simulink model ""  (R2026a)
settings: Solver=FixedStepDiscrete  StopTime=Inf  FixedStep=0.01
PreLoadFcn:
  | rbt = exampleHelperSetUpCobot();
  | 
  | %maxNumOfBoxes = 30;
  | %boxDim = 0.2;
  | %boxPosition = [-0.65 0.45 0.6];
  | 
  | % initSim.m
  | data = readmatrix('boxes.xlsx');  % Now it's a double matrix
  | boxDim = data(1, 2:4);
  | boxPosition = data(1, 6:8);
  | maxNumOfBoxes = length(data(:,1));
  | boxWeight = data(1,5);
  | assignin('base', 'data', data);
  | assignin('base', 'boxDim', boxDim);
  | assignin('base', 'boxPosition', boxPosition);
InitFcn:
  | data = readmatrix('boxes.xlsx');  % Now it's a double matrix
  | boxDim = data(1, 2:4);
  | boxPosition = data(1, 6:8);
  | maxNumOfBoxes = length(data(:,1));
  | boxWeight = data(1,5);
StartFcn:
  | coder.extrinsic("spawnBox")
  | 
  | % Spawn the first box on the bench
  | K = [0.2, 0.2, 0.2];
  | Wt = 0.2;
  | spawnBox(0, boxPosition, boxDim, boxWeight)
libraries: sim3dlib x2, robotcorelib x2, robotmaniplib x2, robotsim3dlib x1
settings Model: PauseTimes=1  Creator=araman  LastModifiedBy=fofr6825
settings DebuggingCC: ReadBeforeWriteMsg=DisableAll  WriteAfterWriteMsg=DisableAll  WriteAfterReadMsg=DisableAll  MultiTaskDSMMsg=none
settings SFSimCC: SFSimEcho=off
settings SimscapeCC: SimscapeNominalValues="[{\"value\":\"1\",\"unit\":\"A\"},{\"value\":\"1\",\"unit\":\"bar\"},{\"value\":\"1\",\"unit\":\"cm^2\"},{\"value\":\"1\",\"unit\":\"cm^3/s\"},{\"value\":\"1\",\"unit\":\"kJ/kg\"},{\"value\":\"1\",\"unit\":\"kW\"},{\"value\":\"1\",\"unit\":\"l\"},{\"value\":\"1\",\"unit\":\"N\"},{\"value\":\"1\",\"unit\":\"N*m\"},{\"value\":\"1\",\"unit\":\"V\"}]"  SimscapeLogType=none  SimscapeLogDataHistory=5000.0

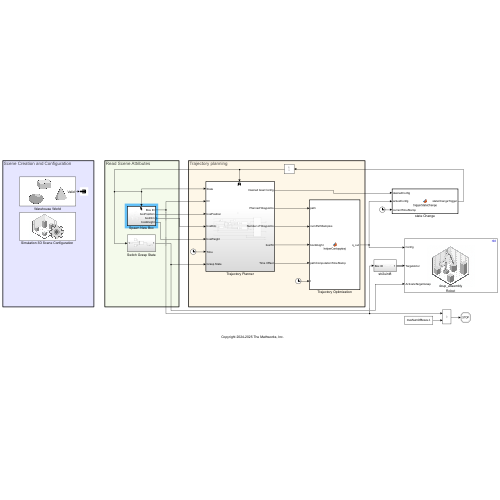
[thumbnail: Simulink's stored preview of the top-level diagram]
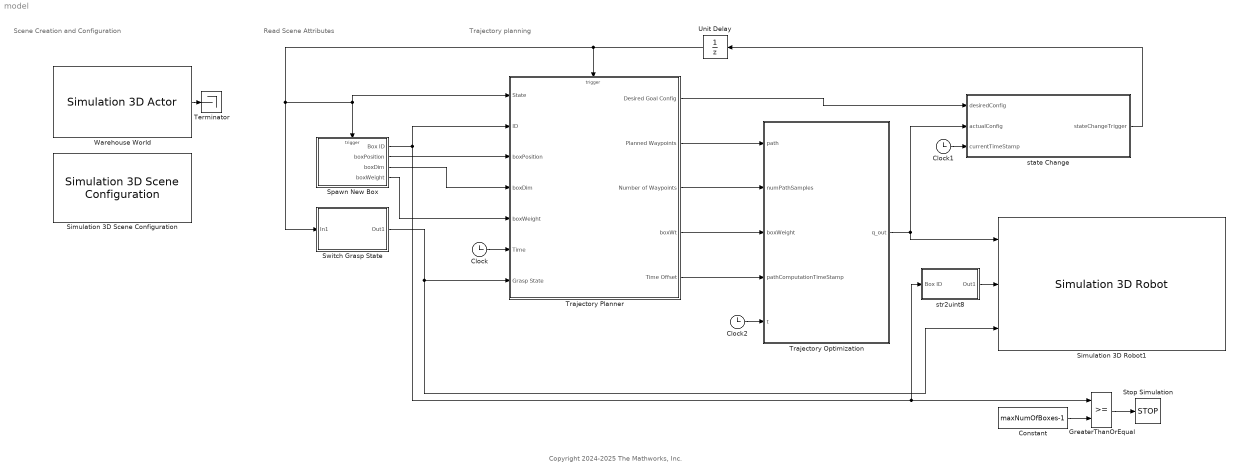
== system model ==
  note: Copyright 2024-2025 The Mathworks, Inc.
  note: Trajectory planning
  note: Scene Creation and Configuration
  note: Read Scene Attributes
  Clock : Clock
  Clock1 : Clock
  Clock2 : Clock
  Constant : Constant  Value=maxNumOfBoxes-1
  GreaterThanOrEqual : RelationalOperator  OutDataTypeStr=boolean  RndMeth=Simplest  InputSameDT=off
  Simulation 3D Robot1 : robotsim3dlib/Simulation 3D Robot  actorInputType=RigidBodyTree Object  RigidBodyTree=rbt  ActorName=Robot  existActorChekBox=off  initialTrans=[0 0 0]  initialRot=[0 0 0]  initialConfig="[2.8471   -1.6598    2.1329    4.2393   -1.5708    4.4179]"  EndEffector=4cup_assembly  eeOffsetInpChekBox=off  eeTargetTrans=[0 -0.2 0]  eeTargetRot=[0 0 0]  enableRegionGraspChekBox=off  regionGraspInpChekBox=off  eeTargTransDiff=[0.2 0.2 0.2]  eeTargRotDiff=[0 0 0]  enableVisualVisualization=on  enableCollisionVisualization=off  collisionGeomColor=[0 1 0]  collisionGeomTransp=0.1  inpConfEnbVal=on  inpGraspEnbVal=on  inpTransEnbVal=off  outConfEnbVal=off  outGraspEnbVal=off  outTransEnbVal=off  SampleTime=-1  ActorType=SimulinkVehicle  ID=C  aMode=6  ActorTag=Robot  Mesh=RigidBodyTree
  "Simulation 3D Scene Configuration " : sim3dlib/Simulation 3D Scene Configuration  Priority=0  ProjectFormat=Default Scenes  SceneDesc=Empty scene  ProjectName=C:\Program Files\MATLAB\R2026a\toolbox\shared\sim3d_projects\automotive_project_windows\UE\WindowsNoEditor\VehicleSimulation.exe  ScenePath=/Game/Maps/EmptyScene  EnableOpenDRIVE=off  vehTagList={'Custom';'Robot';'Scene Origin';'Warehouse'}  vehTag=Robot  AttachedCameraRelativeTranslation=[0 0 0]  FreeCameraDefaultInitialTranslation=[-6, 0, 2]  AttachedCameraRelativeRotation=[0 0 0]  FreeCameraDefaultInitialRotation=[0, -15, 0]  ViewpointName=Custom  FreeCameraInitialTranslation=[0, 0, 5]  FreeCameraInitialRotation=[0, -90, 0]  OpVisEn=off  Ts=0.02  EnableWindow=on  EnableRemoteAccess=off  SimulationMode=CoSimulation  SimulateUsing=Interpreted execution  EnableAnimationRecording=off  OverrideDefaultRecording=off  AnimationRecordingFileName=sim3dAnimation.mat  AnimationRecordingInterval=[0 inf]  EnableWeather=off  SunAzimuth=90  SunAltitude=40.0  EnableGeospatialSun=off  Latitude=0  Longitude=0  Date=2023-01-01  Time=10:30:00  GeoTimeZone=-5.0  SunDaylightSaving=off  wind=1  clouds=10  EnableVolumetricClouds=off  CloudCoverage=0  CloudAltitude=6  fog=0  rain=0  RaindropsEffect=off  SnowDensity=0  EnableGeospatial=off  TilesetSource=Earth terrain  UseTrueOrigin=off  OriginHeight=200  OriginLatitude=40.744652  OriginLongitude=-73.988864  MapStyle=Aerial  AdditionalAssetIDs=[]  UseAdvancedSunSky=off  SolarTime=11  TimeZone=-5  Day=21  Month=9  Year=2022  UseDaylightSavingTime=on  DSTStartDay=10  DSTStartMonth=3  DSTEndDay=3  DSTEndMonth=11  DSTSwitchHour=2  sensorTag=MainCamera2  sensorId=2  sensorName=MainCamera2  mountLoc=Origin  offsetFlag=off  tmountOffset=[0, 0, 0]  rmountOffset=[0, 0, 0]  HorizontalResolution=1280  VerticalResolution=720  HorizontalFOV=60  mountPoint=[0 0 0]  mountOrientation=[0 0 0]  aMode=6  ID=2  GeoTrigger=Inactive  ViewNameList={'Custom'}  ViewTranslationList={'[0 0 5]'}  ViewRotationList={'[0 -90 0]'}
      settings: LibrarySourceBlock=robotsim3dlib/Simulation 3D Scene Configuration
  Spawn New Box : Subsystem  TreatAsAtomicUnit=on
  Stop Simulation : Stop
  Switch Grasp State : Subsystem
  Terminator : Terminator
  Trajectory Optimization : MATLAB Function  TreatAsAtomicUnit=on
  Trajectory Planner : Subsystem
  Unit Delay : UnitDelay  InitialCondition=-1  SampleTime=-1
  Warehouse World : sim3dlib/Simulation 3D Actor  Priority=1  ActorName=Warehouse  ParentName=Scene Origin  Operation=Create at setup  InitScriptText=|  SampleTime=-1  Translation=single([0 0 0])  Rotation=single([0 0 0])  Scale=single([1 1 1])  aMode=5  ActorTag=Warehouse  ActorType=Sim3dActor  ID=2
      | Plane = sim3d.Actor(ActorName='Plane');
      | Plane.createShape('plane',[5 5 0.1]);
      | Plane.PreciseContacts = true;
      | Plane.Color = [81, 94, 120]/256;
      | add(World,Plane,Actor);
      | 
      | Base = sim3d.Actor('ActorName','collBase');
      | Base.createShape('box',[0.25,0.25,0.5]);
      | Base.Translation = [0,0,0.25];
      | Base.Color = [87, 67, 60]/256;
      | add(World,Base,Actor);
      | 
      | Bench = sim3d.Actor('ActorName','collBench');
      | Bench.createShape('box',[0.8 0.8 0.5]);
      | Bench.Translation = [-0.7 -0.7 0.25];
      | Bench.Color = [87, 67, 60]/256;
      | add(World,Bench,Actor);
      | 
      | Pallet = sim3d.Actor(ActorName='collPallet');
      | add(World,Pallet,Actor)
      | load(Pallet,"PalletEuro.stl",0.001*[1 1 1]);
      | Pallet.Translation = [-1.2 -0.1 0];
  state Change : MATLAB Function  TreatAsAtomicUnit=on
  str2uint8 : Subsystem
  wires:
  Warehouse World/1 -> Terminator/1
  Unit Delay/1 -> Trajectory Planner/Trigger, Switch Grasp State/1(In1), Spawn New Box/Trigger, Trajectory Planner/1(State)
  Clock/1 -> Trajectory Planner/6(Time)
  Trajectory Planner/2(Planned Waypoints) -> Trajectory Optimization/1(path)
  Trajectory Planner/3(Number of Waypoints) -> Trajectory Optimization/2(numPathSamples)
  Trajectory Planner/5(Time Offset) -> Trajectory Optimization/4(pathComputationTimeStamp)
  Trajectory Planner/1(Desired Goal Config) -> state Change/1(desiredConfig)
  Spawn New Box/1(Box ID) -> GreaterThanOrEqual/1, str2uint8/1(Box ID), Trajectory Planner/2(ID)
  Clock1/1 -> state Change/3(currentTimeStamp)
  state Change/1(stateChangeTrigger) -> Unit Delay/1
  Clock2/1 -> Trajectory Optimization/5(t)
  Switch Grasp State/1(Out1) -> Simulation 3D Robot1/3, Trajectory Planner/7(Grasp State)
  Trajectory Optimization/1(q_out) -> Simulation 3D Robot1/1, state Change/2(actualConfig)
  Constant/1 -> GreaterThanOrEqual/2
  GreaterThanOrEqual/1 -> Stop Simulation/1
  str2uint8/1(Out1) -> Simulation 3D Robot1/2
  Spawn New Box/2(boxPosition) -> Trajectory Planner/3(boxPosition)
  Spawn New Box/3(boxDim) -> Trajectory Planner/4(boxDim)
  Spawn New Box/4(boxWeight) -> Trajectory Planner/5(boxWeight)
  Trajectory Planner/4(boxWt) -> Trajectory Optimization/3(boxWeight)

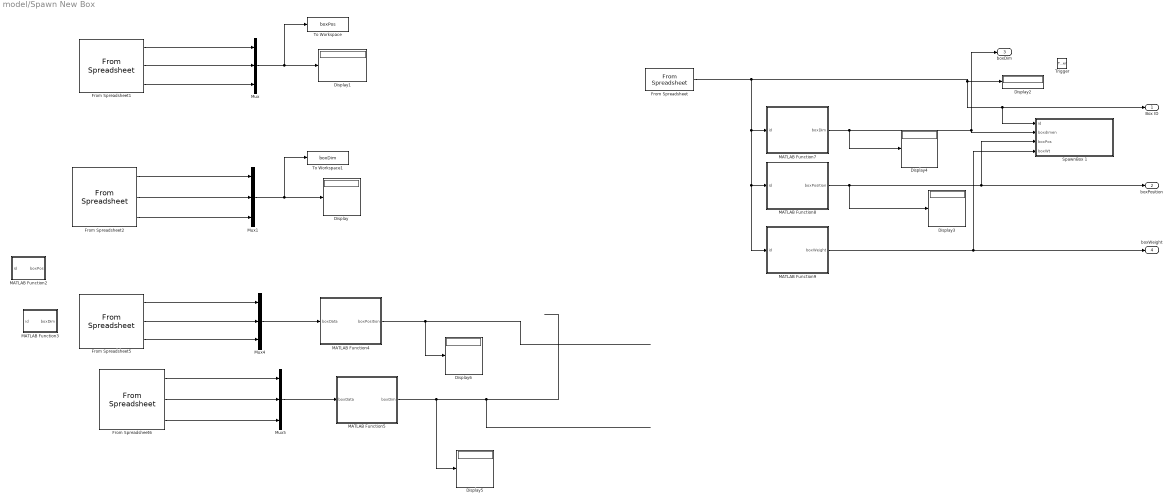
== system model/Spawn New Box ==
  Trigger : TriggerPort  TriggerType=falling  VariantControl=(inherit)
  Display{,1..6} (7 alike) : Display
  From Spreadsheet : FromSpreadsheet  FileName=boxes.xlsx  SheetName=Feuil1  Range=A3:A31  TreatFirstColumnAs=Data  SampleTime=-1  OutputAfterLastPoint=Ground value
  From Spreadsheet1 : FromSpreadsheet  FileName=boxes.xlsx  SheetName=Feuil1  Range=A2:A31, F2:H31  SampleTime=-1
  From Spreadsheet2 : FromSpreadsheet  FileName=boxes.xlsx  SheetName=Feuil1  Range=A2:A31, B2:D31  SampleTime=-1
  From Spreadsheet5 : FromSpreadsheet  FileName=boxes.xlsx  SheetName=Feuil1  Range=F3:H31  TreatFirstColumnAs=Data  SampleTime=-1
  From Spreadsheet6 : FromSpreadsheet  FileName=boxes.xlsx  SheetName=Feuil1  Range=B3:D31  TreatFirstColumnAs=Data  SampleTime=-1
  MATLAB Function2 : MATLAB Function  TreatAsAtomicUnit=on
  MATLAB Function3 : MATLAB Function  TreatAsAtomicUnit=on
  MATLAB Function4 : MATLAB Function  TreatAsAtomicUnit=on
  MATLAB Function5 : MATLAB Function  TreatAsAtomicUnit=on
  MATLAB Function7 : MATLAB Function  TreatAsAtomicUnit=on
  MATLAB Function8 : MATLAB Function  TreatAsAtomicUnit=on
  MATLAB Function9 : MATLAB Function  TreatAsAtomicUnit=on
  Mux{,1,4..5} (4 alike) : Mux  Inputs=3
  SpawnBox 1 : MATLAB Function  TreatAsAtomicUnit=on
  To Workspace : ToWorkspace  VariableName=boxPos  SaveFormat=Timeseries  SampleTime=-1
  To Workspace1 : ToWorkspace  VariableName=boxDim  SaveFormat=Timeseries  SampleTime=-1
  Box ID : Outport
  boxPosition : Outport  Port=2  InitialOutput=boxPosition
  boxDim : Outport  Port=3  InitialOutput=boxDim
  boxWeight : Outport  Port=4  InitialOutput=boxWeight
  wires:
  From Spreadsheet/1 -> SpawnBox 1/1(id), Box ID/1, Display2/1, MATLAB Function9/1(id), MATLAB Function8/1(id), MATLAB Function7/1(id)
  Mux/1 -> To Workspace/1, Display1/1
  From Spreadsheet1/3 -> Mux/3
  From Spreadsheet1/1 -> Mux/1
  From Spreadsheet1/2 -> Mux/2
  Mux1/1 -> To Workspace1/1, Display/1
  From Spreadsheet2/2 -> Mux1/2
  From Spreadsheet2/3 -> Mux1/3
  From Spreadsheet2/1 -> Mux1/1
  MATLAB Function4/1(boxPosition) -> Display6/1
  From Spreadsheet5/3 -> Mux4/3
  From Spreadsheet6/3 -> Mux5/3
  MATLAB Function5/1(boxDim) -> Display5/1
  From Spreadsheet6/1 -> Mux5/1
  Mux5/1 -> MATLAB Function5/1(boxData)
  From Spreadsheet5/1 -> Mux4/1
  From Spreadsheet5/2 -> Mux4/2
  Mux4/1 -> MATLAB Function4/1(boxData)
  From Spreadsheet6/2 -> Mux5/2
  MATLAB Function7/1(boxDim) -> boxDim/1, SpawnBox 1/2(boxdimen), Display4/1
  MATLAB Function8/1(boxPosition) -> Display3/1, boxPosition/1, SpawnBox 1/3(boxPos)
  MATLAB Function9/1(boxWeight) -> boxWeight/1, SpawnBox 1/4(boxWt)

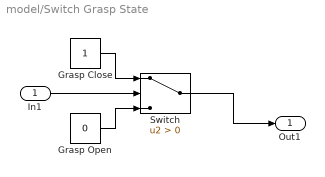
== system model/Switch Grasp State ==
  In1 : Inport
  Grasp Close : Constant  OutDataTypeStr=boolean
  Grasp Open : Constant  Value=0  OutDataTypeStr=boolean
  Switch : Switch  Criteria=u2 > Threshold  SaturateOnIntegerOverflow=off  InputSameDT=off
  Out1 : Outport
  wires:
  Grasp Close/1 -> Switch/1
  Switch/1 -> Out1/1
  Grasp Open/1 -> Switch/3
  In1/1 -> Switch/2

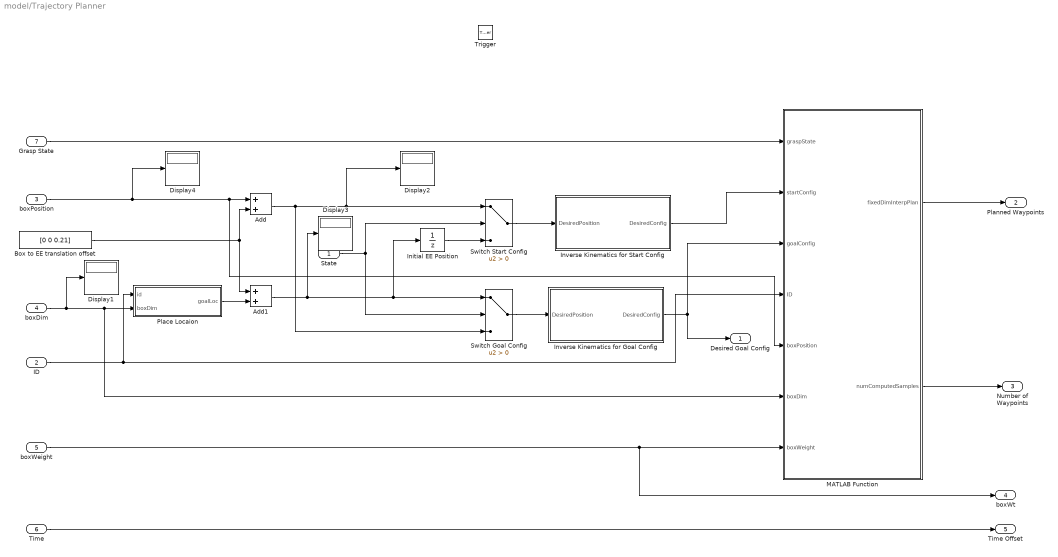
== system model/Trajectory Planner ==
  State : Inport
  ID : Inport  Port=2
  boxPosition : Inport  Port=3
  boxDim : Inport  Port=4
  boxWeight : Inport  Port=5
  Time : Inport  Port=6
  Grasp State : Inport  Port=7
  Trigger : TriggerPort  TriggerType=either  VariantControl=(inherit)  OutputDataType=double  InitialTriggerSignalState=zero  PortDimensions=1
  Add : Sum
  Add1 : Sum
  Box to EE translation offset : Constant  Value=[0 0 0.21]  VectorParams1D=off
  Display{1..4} (4 alike) : Display
  Initial EE Position : UnitDelay  InitialCondition=[-0.6 0 0.8]  SampleTime=-1
  Inverse Kinematics for Goal Config : Subsystem
  Inverse Kinematics for Start Config : Subsystem
  MATLAB Function : MATLAB Function  TreatAsAtomicUnit=on
  Place Locaion : MATLAB Function  TreatAsAtomicUnit=on
  Switch Goal Config : Switch  Criteria=u2 > Threshold  SaturateOnIntegerOverflow=off  InputSameDT=off
  Switch Start Config : Switch  Criteria=u2 > Threshold  SaturateOnIntegerOverflow=off  InputSameDT=off
  Desired Goal Config : Outport
  Planned Waypoints : Outport  Port=2
  Number of Waypoints : Outport  Port=3
  boxWt : Outport  Port=4  InitialOutput=boxWeight
  Time Offset : Outport  Port=5
  wires:
  MATLAB Function/1(fixedDimInterpPlan) -> Planned Waypoints/1
  MATLAB Function/2(numComputedSamples) -> Number of Waypoints/1
  Inverse Kinematics for Start Config/1(DesiredConfig) -> MATLAB Function/2(startConfig)
  Inverse Kinematics for Goal Config/1(DesiredConfig) -> MATLAB Function/3(goalConfig), Desired Goal Config/1
  Time/1 -> Time Offset/1
  Switch Start Config/1 -> Inverse Kinematics for Start Config/1(DesiredPosition)
  Initial EE Position/1 -> Switch Start Config/3
  Switch Goal Config/1 -> Inverse Kinematics for Goal Config/1(DesiredPosition)
  State/1 -> Switch Start Config/2, Switch Goal Config/2
  Grasp State/1 -> MATLAB Function/1(graspState)
  ID/1 -> MATLAB Function/4(ID), Place Locaion/1(id)
  Place Locaion/1(goalLoc) -> Add1/2
  Box to EE translation offset/1 -> Add1/1, Add/2
  Add1/1 -> Initial EE Position/1, Switch Goal Config/1, Display3/1
  boxDim/1 -> Display1/1, MATLAB Function/6(boxDim), Place Locaion/2(boxDim)
  boxPosition/1 -> Display4/1, MATLAB Function/5(boxPosition), Add/1
  boxWeight/1 -> boxWt/1, MATLAB Function/7(boxWeight)
  Add/1 -> Display2/1, Switch Start Config/1, Switch Goal Config/3

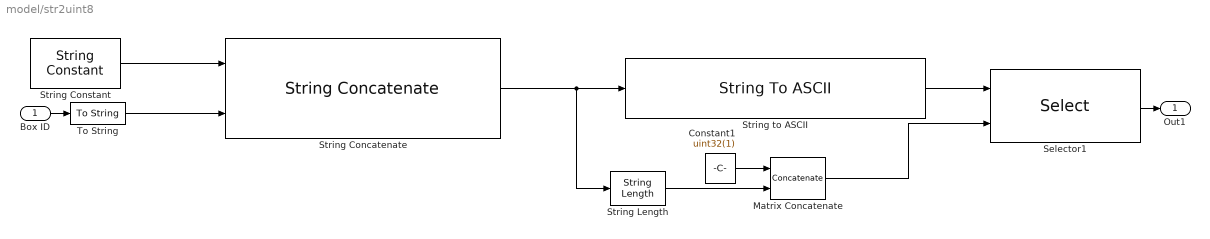
== system model/str2uint8 ==
  Box ID : Inport
  Constant1 : Constant  Value=uint32(1)
  Matrix Concatenate : Concatenate  ConcatenateDimension=2
  Selector1 : Selector  InputPortWidth=12  IndexOptions=Starting and ending indices (port)  Indices=[1 3]  OutputSizes=1
  String Concatenate : StringConcatenate
  String Constant : StringConstant  String="\"collBox\""
  String Length : StringLength
  String to ASCII : StringToASCII  OutputVectorSize=12
  To String : ToString
  Out1 : Outport
  wires:
  String Constant/1 -> String Concatenate/1
  Constant1/1 -> Matrix Concatenate/1
  String Length/1 -> Matrix Concatenate/2
  String Concatenate/1 -> String Length/1, String to ASCII/1
  Box ID/1 -> To String/1
  Matrix Concatenate/1 -> Selector1/2
  String to ASCII/1 -> Selector1/1
  To String/1 -> String Concatenate/2
  Selector1/1 -> Out1/1

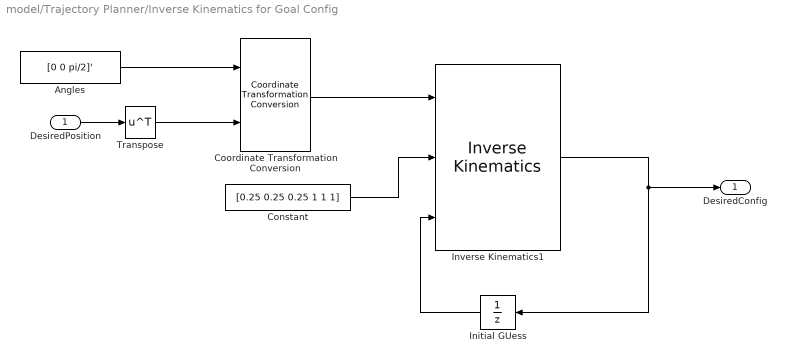
== system model/Trajectory Planner/Inverse Kinematics for Goal Config ==
  DesiredPosition : Inport
  Angles : Constant  Value=[0 0 pi/2]'  VectorParams1D=off
  Constant : Constant  Value=[0.25 0.25 0.25 1 1 1]
  Coordinate Transformation Conversion : robotcorelib/Coordinate Transformation Conversion  InputRepresentation=Euler Angles  InputEulerSequence=ZYX  ShowTrVecInputPort=on  OutputRepresentation=Homogeneous Transformation  OutputEulerSequence=ZYX  ShowTrVecOutputPort=on  SimulateUsing=Interpreted execution
  Initial GUess : UnitDelay  InitialCondition="[2.8471   -1.6598    2.1329    4.2393   -1.5708    4.4179]'"  SampleTime=-1
  Inverse Kinematics1 : robotmaniplib/Inverse Kinematics  RigidBodyTree=rbt  EndEffector=4cup_assembly  ShowInfo=off  SolverName=BFGS Gradient Projection  EnforceJointLimits=on  AllowRandomRestarts=off  MaxIterations=40  MaxTime=10  GradientTolerance=1e-7  SolutionTolerance=1e-6  StepTolerance=1e-14  ConstraintTolerance=1e-6  ErrorChangeTolerance=1e-12  UseErrorDamping=on  DampingBias=0.0025  RandomStream=Global stream  Seed=0  SimulateUsing=Code generation
  Transpose : Math  Operator=transpose
  DesiredConfig : Outport
  wires:
  Constant/1 -> Inverse Kinematics1/2
  Angles/1 -> Coordinate Transformation Conversion/1
  Coordinate Transformation Conversion/1 -> Inverse Kinematics1/1
  DesiredPosition/1 -> Transpose/1
  Initial GUess/1 -> Inverse Kinematics1/3
  Inverse Kinematics1/1 -> Initial GUess/1, DesiredConfig/1
  Transpose/1 -> Coordinate Transformation Conversion/2

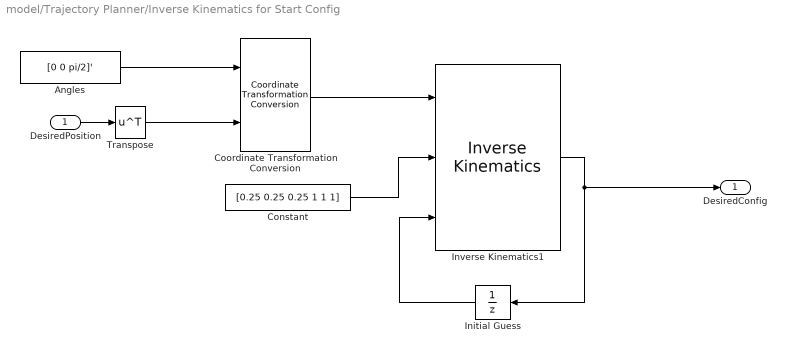
== system model/Trajectory Planner/Inverse Kinematics for Start Config ==
  DesiredPosition : Inport
  Angles : Constant  Value=[0 0 pi/2]'  VectorParams1D=off
  Constant : Constant  Value=[0.25 0.25 0.25 1 1 1]
  Coordinate Transformation Conversion : robotcorelib/Coordinate Transformation Conversion  InputRepresentation=Euler Angles  InputEulerSequence=ZYX  ShowTrVecInputPort=on  OutputRepresentation=Homogeneous Transformation  OutputEulerSequence=ZYX  ShowTrVecOutputPort=on  SimulateUsing=Interpreted execution
  Initial Guess : UnitDelay  InitialCondition="[-0.0724   -0.8022    1.6836    3.8   -1.5708    1.3514]'"  SampleTime=-1
  Inverse Kinematics1 : robotmaniplib/Inverse Kinematics  RigidBodyTree=rbt  EndEffector=4cup_assembly  ShowInfo=off  SolverName=BFGS Gradient Projection  EnforceJointLimits=on  AllowRandomRestarts=off  MaxIterations=40  MaxTime=10  GradientTolerance=1e-7  SolutionTolerance=1e-6  StepTolerance=1e-14  ConstraintTolerance=1e-6  ErrorChangeTolerance=1e-12  UseErrorDamping=on  DampingBias=0.0025  RandomStream=Global stream  Seed=0  SimulateUsing=Code generation
  Transpose : Math  Operator=transpose
  DesiredConfig : Outport
  wires:
  Constant/1 -> Inverse Kinematics1/2
  Angles/1 -> Coordinate Transformation Conversion/1
  Inverse Kinematics1/1 -> DesiredConfig/1, Initial Guess/1
  Initial Guess/1 -> Inverse Kinematics1/3
  Coordinate Transformation Conversion/1 -> Inverse Kinematics1/1
  DesiredPosition/1 -> Transpose/1
  Transpose/1 -> Coordinate Transformation Conversion/2

== matlab function Spawn New Box/MATLAB Function7 ==
  data: id input; boxDim output
function boxDim = getBoxDim(id)
coder.extrinsic('evalin');
data = zeros(30,8);              % known type/size before extrinsic call
data = evalin('base','data');
boxDim = double(data(id+1, 2:4));
boxDim = reshape(boxDim, 1, 3);
end

== matlab function Spawn New Box/MATLAB Function8 ==
  data: id input; boxPosition output
function boxPosition = getBoxPosition(id)
coder.extrinsic('evalin');
data = zeros(30,8);
data = evalin('base','data');
boxPosition = double(data(id+1, 6:8));
boxPosition = reshape(boxPosition, 1,3);
end

== matlab function Spawn New Box/MATLAB Function9 ==
  data: id input; boxWeight output
function boxWeight = getBoxWeight(id)
coder.extrinsic('evalin');
data = zeros(30,8);
data = evalin('base','data');
boxWeight = double(data(id+1, 5));
end

== matlab function Trajectory Planner/MATLAB Function ==
  data: graspState input; startConfig input; fixedDimInterpPlan output size=[6,200]; goalConfig input; ID input; boxPosition input; boxDim input; boxWeight input; numComputedSamples output; maxNumOfBoxes parameter
function [fixedDimInterpPlan,numComputedSamples] = helperPathPanning(graspState, startConfig,goalConfig,ID,boxPosition, boxDim, boxWeight, maxNumOfBoxes)
% Declare extrinsic at top-level
coder.extrinsic('exampleHelperManipulatorRRT');

% Define fixed output types/sizes for codegen
NUMDOF = 6;
NUMPATHSAMPLES = 200;
fixedDimInterpPlan = zeros(NUMDOF, NUMPATHSAMPLES); % double
numComputedSamples = double(0);                       % integer
[fixedDimInterpPlan, numComputedSamples] = exampleHelperManipulatorRRT(graspState, startConfig,goalConfig,ID,boxPosition, boxDim, boxWeight, maxNumOfBoxes);
end

== matlab function state Change ==
  data: desiredConfig input; stateChangeTrigger output; actualConfig input; currentTimeStamp input
function stateChangeTrigger = triggerStateChange(desiredConfig,actualConfig, currentTimeStamp)

tol = sqrt(eps);
simTimeStep = 0.01; % discrete time step of the simulation

persistent stateChange timeAtStateChange
if isempty(stateChange)
    stateChange = -1;
    timeAtStateChange = 0;
end

% Ensure that the goal position is reached and held for at least one
% simulation time step
if sqrt(sum((desiredConfig-actualConfig).^2)) < tol && (currentTimeStamp - timeAtStateChange) > simTimeStep
    switch stateChange
        case -1 
            stateChange = 1;
        case 1
            stateChange = -1; 
    end
    timeAtStateChange = currentTimeStamp;
end

stateChangeTrigger = stateChange;

end

== matlab function Trajectory Optimization ==
  data: path input size=[6,200]; numPathSamples input; boxWeight input; pathComputationTimeStamp input; t input; q_out output
function q_out = helperContopptraj(path, numPathSamples, boxWeight, pathComputationTimeStamp, t)

% Nominal (empty-gripper) joint velocity/acceleration limits
VELLIM_NOM   = repmat([-10  10], 6, 1);   % rad/s
ACCELLIM_NOM = repmat([-15  15], 6, 1);   % rad/s^2

% Payload-based derating: heavier box -> lower speed/accel limits
maxPayload = 12.5;   % kg, UR10e rated payload — adjust to your gripper's actual capacity
minScale   = 0.4;    % never drop below 40% speed, even at max rated payload
payloadFrac = min(max(double(boxWeight),0) / maxPayload, 1);
speedScale  = 1 - (1 - minScale) * payloadFrac;

VELLIM   = VELLIM_NOM   * speedScale;
ACCELLIM = ACCELLIM_NOM * speedScale;

% Store the last time at which the path was computed as a persistent
% variable. This allows the function to detect changes
persistent prevPathComputationTime qSolve tSolve
if isempty(prevPathComputationTime)
    prevPathComputationTime = -1;
end
if isempty(qSolve)
    qSolve = repmat([2.8471   -1.6598    2.1329    4.2393   -1.5708    4.4179]',1,500);
    tSolve = linspace(0,2,500);
end
% Compute a time constrained trajectory with contoptraj
if (pathComputationTimeStamp ~= prevPathComputationTime) && (numPathSamples > 0)
    [qSolve,~,~,tSolve] = contopptraj(path(:,1:numPathSamples),VELLIM,ACCELLIM,NumSamples=100);
end
q_out = zeros(6,1);
maxTime = max(tSolve);
queryTime = t - pathComputationTimeStamp;
if queryTime == 0
    q_out(:) = qSolve(:,1);
elseif queryTime <= maxTime
    q_out(:) = interp1(tSolve,qSolve',queryTime);
else
    q_out(:) = qSolve(:,end);
end
prevPathComputationTime = pathComputationTimeStamp;
end

== matlab function Spawn New Box/SpawnBox 1 ==
  data: id input; boxdimen input; boxPos input; boxWt input
function spawnBoxOnBench(id,boxdimen, boxPos, boxWt)
 boxPosition = reshape(boxPos, 1,3);
 boxDim = reshape(boxdimen, 1,3);
 boxWeight = double(boxWt);
 coder.extrinsic("spawnBox")
 spawnBox(id,boxPosition,boxDim,boxWeight)
end

== matlab function Spawn New Box/MATLAB Function2 ==
  data: id input; boxPos output
function boxPos = getBoxPosition(id)
%GETBOXPOSITION Look up the pick position [X Y Z] for a given box id.
%   boxPos = getBoxPosition(id) reads boxes.xlsx (columns pickX, pickY,
%   pickZ) and returns the 1x3 position row for the box whose id matches
%   the input. id=0 -> spreadsheet row 1, id=1 -> row 2, etc.

coder.extrinsic('readmatrix');

persistent data
if isempty(data)
    data = zeros(30,8);            % preallocate: readmatrix auto-drops the header row
    data = readmatrix('boxes.xlsx');
end

if isnan(id)
    boxPos = [-0.65 0.45 0.6];     % known-safe default, matches your test constant
    return
end

row = round(double(id)) + 1;
row = min(max(row,1), size(data,1));   % clamp to a valid row

boxPos = reshape(double(data(row,6:8)),1,3);   % pickX, pickY, pickZ
end

== matlab function Spawn New Box/MATLAB Function3 ==
  data: id input; boxDim output
function boxDim = getBoxDim(id)
%GETBOXDIM Look up the dimensions [Length Width Height] for a given box id.
%   boxDim = getBoxDim(id) reads boxes.xlsx (columns Length, width,
%   Height) and returns the 1x3 dimension row for the box whose id
%   matches the input. id=0 -> spreadsheet row 1, id=1 -> row 2, etc.
coder.extrinsic('readmatrix');
persistent data
if isempty(data)
    data = zeros(30,8);            % preallocate: readmatrix auto-drops the header row
    data = readmatrix('boxes.xlsx');
end

if isnan(id)
    boxDim = [0.2 0.2 0.2];        % known-safe default, matches your test constant
    return
end

row = round(double(id)) + 1;
row = min(max(row,1), size(data,1));   % clamp to a valid row

boxDim = reshape(double(data(row,2:4)),1,3);   % Length, width, Height
end

== matlab function Trajectory Planner/Place Locaion ==
  data: id input; goalLoc output; boxDim input
function goalLoc = getGoalOnPallet(id, boxDim)
coder.extrinsic("exampleHelperGetInitActorProp")
persistent palletDim palletLoc 
if isempty(palletDim)
    palletLoc = zeros(1,3);
    palletDim = zeros(1,3);
    [~,~,~,~,palletLoc,palletDim] = exampleHelperGetInitActorProp();
end

% Get the positions and dimension of other actors
goalLoc = zeros(1,3);
goalLoc = exampleHelperPalletArrangement(id,palletDim,palletLoc,boxDim);
end

== matlab function Spawn New Box/MATLAB Function4 ==
  data: boxData input; boxPosition output
function boxPosition = getBoxPosition(boxData)
    boxPosition = boxData;
    boxPosition = reshape(double(boxPosition),1,3);
end

== matlab function Spawn New Box/MATLAB Function5 ==
  data: boxData input; boxDim output
function boxDim = getBoxDim(boxData)
    boxDim = boxData;
    boxDim = reshape(double(boxDim),1,3);
end
